simulink model "zd2808_foc_demo"  (R2025b)
settings: Solver=FixedStepDiscrete  StartTime=0.0  StopTime=.42  FixedStep=foc_ts  RelTol=1e-3
PostLoadFcn:
  | addpath(fileparts(fileparts(get_param(bdroot,'FileName'))));balance_setup;
model workspace (MAT data in the model file):
  foc_config = [7 0.09 2.4e-05 2.4e-05 0.00112516101106 2.99678899841e-05 1e-05 7.4 4e-05 0.0753982236862 0.0753982236862 282.743338823 6 10 1]
  foc_ts = 4e-05
settings Model: Creator=16004  LastModifiedBy=16004
settings DataIOCC: SignalLogging=off

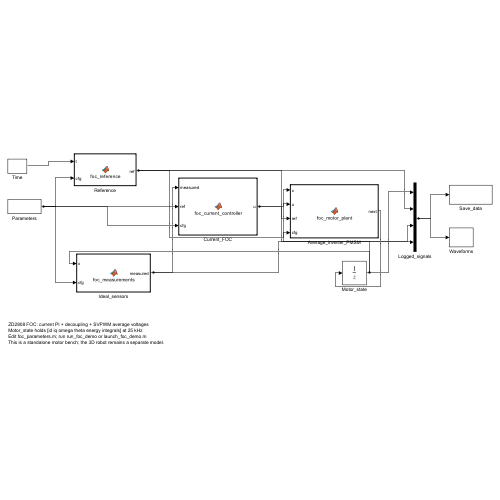
[thumbnail: Simulink's stored preview of the top-level diagram]
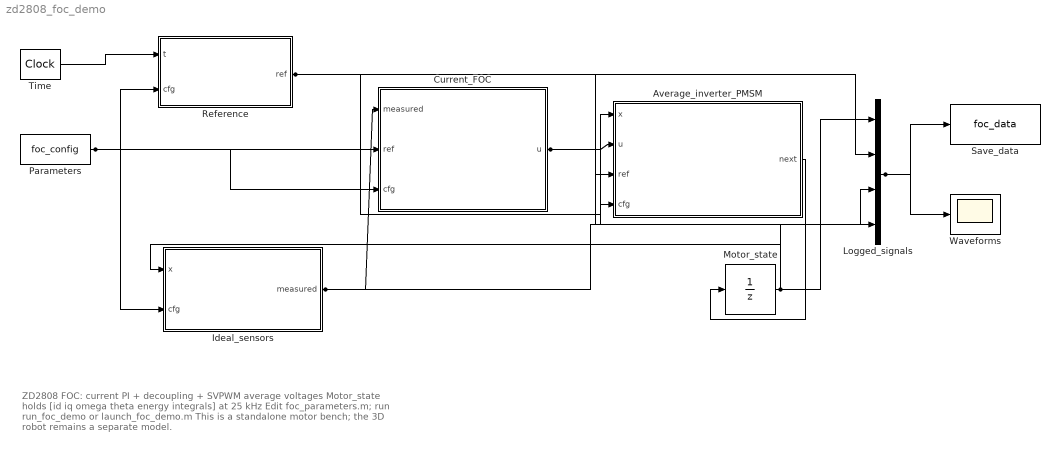
== system zd2808_foc_demo ==
  note: ZD2808 FOC: current PI + decoupling + SVPWM average voltages
      | Motor_state holds [id iq omega theta energy integrals] at 25 kHz
      | Edit foc_parameters.m; run run_foc_demo or launch_foc_demo.m
      | This is a standalone motor bench; the 3D robot remains a separate model.
  Average_inverter_PMSM : MATLAB Function  TreatAsAtomicUnit=on
  Current_FOC : MATLAB Function  TreatAsAtomicUnit=on
  Ideal_sensors : MATLAB Function  TreatAsAtomicUnit=on
  Logged_signals : Mux
  Motor_state : UnitDelay  InitialCondition=zeros(7,1)  SampleTime=foc_ts  HasFrameUpgradeWarning=on
  Parameters : Constant  Value=foc_config
  Reference : MATLAB Function  TreatAsAtomicUnit=on
  Save_data : ToWorkspace  VariableName=foc_data  SaveFormat=Timeseries  SampleTime=-1
  Time : DigitalClock  SampleTime=foc_ts
  Waveforms : Scope
  wires:
  Time/1 -> Reference/1(t)
  Parameters/1 -> Reference/2(cfg), Ideal_sensors/2(cfg), Current_FOC/3(cfg), Average_inverter_PMSM/4(cfg)
  Motor_state/1 -> Ideal_sensors/1(x), Average_inverter_PMSM/1(x), Logged_signals/1
  Ideal_sensors/1(measured) -> Current_FOC/1(measured), Logged_signals/4
  Reference/1(ref) -> Current_FOC/2(ref), Average_inverter_PMSM/3(ref), Logged_signals/2
  Current_FOC/1(u) -> Average_inverter_PMSM/2(u), Logged_signals/3
  Average_inverter_PMSM/1(next) -> Motor_state/1
  Logged_signals/1 -> Save_data/1, Waveforms/1

== matlab function zd2808_foc_demo/Current_FOC ==
  data: measured input; u output; ref input; cfg input
function u=foc_current_controller(measured,ref,cfg)
%#codegen
% Clarke/Park -> dq PI+解耦 -> 圆形电压限幅 -> SVPWM平均占空比。
persistent integral
if isempty(integral),integral=zeros(2,1);end
alpha=(2*measured(1)-measured(2)-measured(3))/3;
beta=(measured(2)-measured(3))/sqrt(3);
c=cos(measured(4));s=sin(measured(4));
id=c*alpha+s*beta;iq=-s*alpha+c*beta;
iqref=min(max(ref(2),-cfg(13)),cfg(13));error=[ref(1)-id;iqref-iq];
we=cfg(1)*measured(5);
ff=[-we*cfg(4)*iq;we*(cfg(3)*id+cfg(5))];
unsat=[cfg(10)*error(1);cfg(11)*error(2)]+integral+ff;
vmax=cfg(8)/sqrt(3);scale=min(1,vmax/max(norm(unsat),1e-12));vdq=unsat*scale;
% 反算抗积分饱和：回算时间常数采用Ld/Rs。
kaw=cfg(12)/cfg(10);
integral=integral+cfg(9)*(cfg(12)*error+kaw*(vdq-unsat));
va=c*vdq(1)-s*vdq(2);vb=s*vdq(1)+c*vdq(2);
phase=[va;-.5*va+sqrt(3)/2*vb;-.5*va-sqrt(3)/2*vb];
common=-(max(phase)+min(phase))/2;
duty=.5+(phase+common)/cfg(8);duty=min(max(duty,0),1);
% 两电平逆变器的平均相电压，去除浮动中性点共模。
applied=cfg(8)*(duty-sum(duty)/3);
ab=[(2*applied(1)-applied(2)-applied(3))/3;(applied(2)-applied(3))/sqrt(3)];
% u=[v_alpha v_beta vd vq dutyA dutyB dutyC saturated iq_limited]。
u=[ab;vdq;duty;double(scale<1-1e-9);iqref];
end

== matlab function zd2808_foc_demo/Reference ==
  data: t input; ref output; cfg input
function ref=foc_reference(t,cfg)
%#codegen
% ref=[id指令 iq原始指令 外负载转矩 锁轴标志]。
iq=0;load=0;locked=0;scenario=round(cfg(15));
if scenario==1
 locked=1;
 if t>=.02&&t<.10,iq=2;
 elseif t>=.10&&t<.18,iq=4;
 elseif t>=.18&&t<.26,iq=-3;
 elseif t>=.26&&t<.34,iq=8;end
elseif scenario==2
 if t>=.02&&t<.20,iq=3;
 elseif t>=.20&&t<.60,iq=-3;end
elseif scenario==3
 if t>=.02,iq=2;end
 if t>=.15&&t<.35,load=.020;end
else
 if t>=.02,iq=6;end
end
ref=[0;iq;load;locked];
end

== matlab function zd2808_foc_demo/Average_inverter_PMSM ==
  data: x input; u input; next output; ref input; cfg input
function next=foc_motor_plant(x,u,ref,cfg)
%#codegen
% x=[id iq omega_mechanical theta_mechanical Ein Ecu Eload]。
% 一个控制周期内保持逆变器alpha/beta平均电压，RK4积分电磁与机械方程。
next=x;h=cfg(9)/cfg(14);
for k=1:round(cfg(14))
 a=derivative(next,u,ref,cfg);
 b=derivative(next+h*a/2,u,ref,cfg);
 c=derivative(next+h*b/2,u,ref,cfg);
 d=derivative(next+h*c,u,ref,cfg);
 next=next+h*(a+2*b+2*c+d)/6;
end
end
function dx=derivative(x,u,ref,cfg)
p=cfg(1);R=cfg(2);Ld=cfg(3);Lq=cfg(4);flux=cfg(5);
id=x(1);iq=x(2);w=x(3);theta=p*x(4);we=p*w;
vd=cos(theta)*u(1)+sin(theta)*u(2);
vq=-sin(theta)*u(1)+cos(theta)*u(2);
torque=1.5*p*(flux*iq+(Ld-Lq)*id*iq);
dx=zeros(7,1);
dx(1)=(vd-R*id+we*Lq*iq)/Ld;
dx(2)=(vq-R*iq-we*(Ld*id+flux))/Lq;
if ref(4)<.5
 dx(3)=(torque-ref(3)-cfg(7)*w)/cfg(6);dx(4)=w;
end
dx(5)=1.5*(vd*id+vq*iq);
dx(6)=1.5*R*(id*id+iq*iq);
dx(7)=(ref(3)+cfg(7)*w)*w;
end

== matlab function zd2808_foc_demo/Ideal_sensors ==
  data: x input; measured output; cfg input
function measured=foc_measurements(x,cfg)
%#codegen
% 理想相电流与转子角度测量。幅值不变逆Park及逆Clarke。
theta=cfg(1)*x(4);c=cos(theta);s=sin(theta);
alpha=c*x(1)-s*x(2);beta=s*x(1)+c*x(2);
measured=[alpha;-.5*alpha+sqrt(3)/2*beta;-.5*alpha-sqrt(3)/2*beta;theta;x(3)];
end
